simulink model "pd_to_wheel_main"  (R2026a)
settings: Solver=ode45  StopTime=200  MaxStep=0.1
settings Model: Creator=user  LastModifiedBy=user

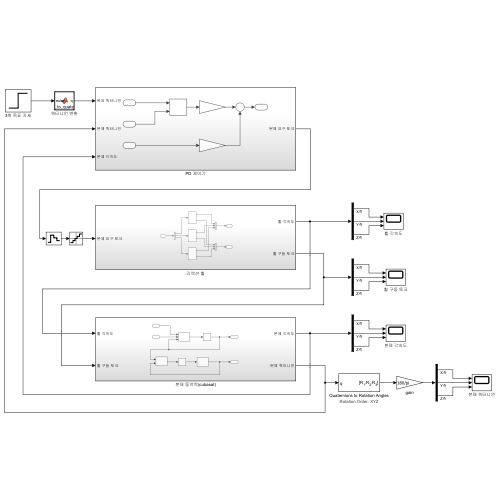
[thumbnail: Simulink's stored preview of the top-level diagram]
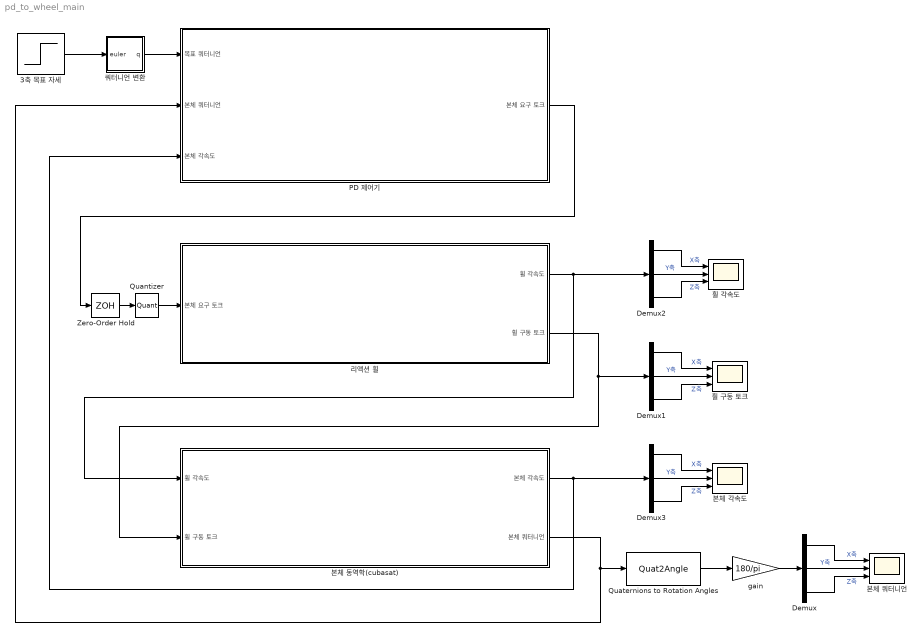
== system pd_to_wheel_main ==
  3축 목표 자세 : Step  InitialValue=[0 0 0]  FinalValue=[5 7 10]*pi/180  SampleTime=0
  Demux{,1..3} (4 alike) : Demux  Outputs=3
  PD 제어기 : Subsystem
  Quantizer : Quantizer  QuantizationInterval=1e-6
  Quaternions to Rotation Angles : Quat2Angle  rotationOrder=XYZ
      settings: AttributesFormatString=Rotation Order: %<rotationOrder>
  Zero-Order Hold : ZeroOrderHold  SampleTime=0.2
  gain : Gain  Gain=180/pi
  리액션 휠 : Subsystem
  본체 각속도 : Scope  NumInputPorts=3
      settings: Title=본체 각속도  ActiveDisplayYMinimum=-0.0017526510151267547  ActiveDisplayYMaximum=0.013773859136141228  DataLoggingVariableName=ScopeData2
  본체 동역학(cubasat) : Subsystem
  본체 쿼터니언 : Scope  NumInputPorts=3
      settings: Title=본체 쿼터니언  ActiveDisplayYMinimum=-1.2703380889069451  ActiveDisplayYMaximum=11.433042800162507
  쿼터니언 변환 : MATLAB Function  TreatAsAtomicUnit=on
  휠 각속도 : Scope  NumInputPorts=3
      settings: Title=휠 가속도  ActiveDisplayYMinimum=-126.21690123764748  ActiveDisplayYMaximum=16.06955468297053
  휠 구동 토크 : Scope  NumInputPorts=3
      settings: Title=휠 구동 토크  ActiveDisplayYMinimum=-0.000403851479395905  ActiveDisplayYMaximum=0.000120427912021545  DataLoggingVariableName=ScopeData3
  wires:
  Zero-Order Hold/1 -> Quantizer/1
  PD 제어기/1(본체 요구 토크) -> Zero-Order Hold/1
  리액션 휠/2(휠 구동 토크) -> Demux1/1, 본체 동역학(cubasat)/2(휠 구동 토크)
  본체 동역학(cubasat)/1(본체 각속도) -> Demux3/1, PD 제어기/3(본체 각속도)
  본체 동역학(cubasat)/2(본체 쿼터니언) -> Quaternions to Rotation Angles/1, PD 제어기/2(본체 쿼터니언)
  Quantizer/1 -> 리액션 휠/1(본체 요구 토크)
  3축 목표 자세/1 -> 쿼터니언 변환/1(euler)
  쿼터니언 변환/1(q) -> PD 제어기/1(목표 쿼터니언)
  리액션 휠/1(휠 각속도) -> Demux2/1, 본체 동역학(cubasat)/1(휠 각속도)
  Quaternions to Rotation Angles/1 -> gain/1
  gain/1 -> Demux/1
  Demux/1 -> 본체 쿼터니언/1  "X축"
  Demux/2 -> 본체 쿼터니언/2  "Y축"
  Demux/3 -> 본체 쿼터니언/3  "Z축"
  Demux1/3 -> 휠 구동 토크/3  "Z축"
  Demux1/2 -> 휠 구동 토크/2  "Y축"
  Demux1/1 -> 휠 구동 토크/1  "X축"
  Demux2/1 -> 휠 각속도/1  "X축"
  Demux2/2 -> 휠 각속도/2  "Y축"
  Demux2/3 -> 휠 각속도/3  "Z축"
  Demux3/3 -> 본체 각속도/3  "Z축"
  Demux3/2 -> 본체 각속도/2  "Y축"
  Demux3/1 -> 본체 각속도/1  "X축"

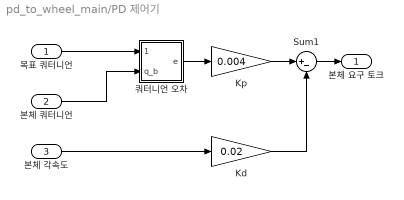
== system pd_to_wheel_main/PD 제어기 ==
  목표 쿼터니언 : Inport  PortDimensions=4
  본체 쿼터니언 : Inport  Port=2  PortDimensions=4
  본체 각속도 : Inport  Port=3  PortDimensions=3
  Kd : Gain  Gain=0.02
  Kp : Gain  Gain=0.004
  Sum1 : Sum  Inputs=|+-
  쿼터니언 오차 : MATLAB Function  TreatAsAtomicUnit=on
  본체 요구 토크 : Outport  PortDimensions=3
  wires:
  Kd/1 -> Sum1/2
  Kp/1 -> Sum1/1
  본체 각속도/1 -> Kd/1
  Sum1/1 -> 본체 요구 토크/1
  쿼터니언 오차/1(e) -> Kp/1
  목표 쿼터니언/1 -> 쿼터니언 오차/1(q_ref)
  본체 쿼터니언/1 -> 쿼터니언 오차/2(q_b)

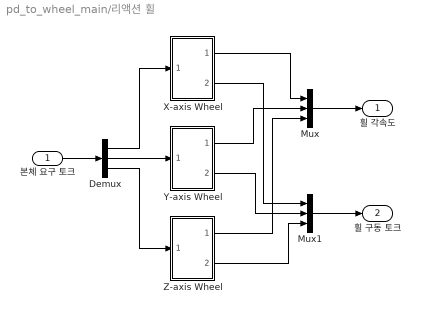
== system pd_to_wheel_main/리액션 휠 ==
  본체 요구 토크 : Inport
  Demux : Demux  Outputs=3
  Mux : Mux  Inputs=3
  Mux1 : Mux  Inputs=3
  X-axis Wheel : Subsystem
  Y-axis Wheel : Subsystem
  Z-axis Wheel : Subsystem
  휠 각속도 : Outport
  휠 구동 토크 : Outport  Port=2
  wires:
  본체 요구 토크/1 -> Demux/1
  Demux/1 -> X-axis Wheel/1(In1)
  Demux/2 -> Y-axis Wheel/1(In1)
  Demux/3 -> Z-axis Wheel/1(In1)
  X-axis Wheel/1(휠 각속도) -> Mux/1
  Y-axis Wheel/1(휠 각속도) -> Mux/2
  Z-axis Wheel/1(휠 각속도) -> Mux/3
  X-axis Wheel/2(휠 구동 토크) -> Mux1/1
  Y-axis Wheel/2(휠 구동 토크) -> Mux1/2
  Z-axis Wheel/2(휠 구동 토크) -> Mux1/3
  Mux/1 -> 휠 각속도/1
  Mux1/1 -> 휠 구동 토크/1

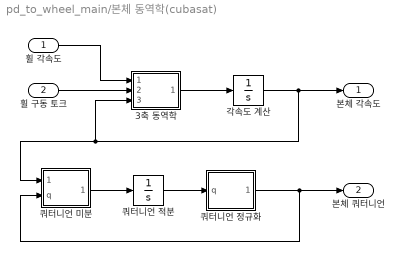
== system pd_to_wheel_main/본체 동역학(cubasat) ==
  휠 각속도 : Inport  PortDimensions=3
  휠 구동 토크 : Inport  Port=2  PortDimensions=3
  3축 동역학 : MATLAB Function  TreatAsAtomicUnit=on
  각속도 계산 : Integrator  InitialCondition=[0;0;0]
  쿼터니언 미분 : MATLAB Function  TreatAsAtomicUnit=on
  쿼터니언 적분 : Integrator  InitialCondition=[1;0;0;0]
  쿼터니언 정규화 : MATLAB Function  TreatAsAtomicUnit=on
  본체 각속도 : Outport  PortDimensions=3
  본체 쿼터니언 : Outport  Port=2  PortDimensions=4
  wires:
  각속도 계산/1 -> 본체 각속도/1, 3축 동역학/3(omega_b), 쿼터니언 미분/1(omega_b)
  휠 각속도/1 -> 3축 동역학/1(omega_w)
  휠 구동 토크/1 -> 3축 동역학/2(tau_w)
  3축 동역학/1(omega_dot) -> 각속도 계산/1
  쿼터니언 미분/1(q_dot) -> 쿼터니언 적분/1
  쿼터니언 적분/1 -> 쿼터니언 정규화/1(q)
  쿼터니언 정규화/1(q_out) -> 쿼터니언 미분/2(q), 본체 쿼터니언/1

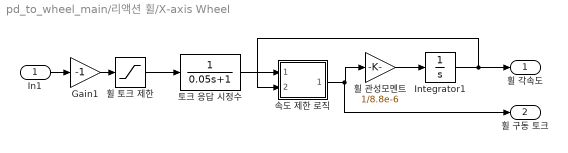
== system pd_to_wheel_main/리액션 휠/X-axis Wheel ==
  In1 : Inport
  Gain1 : Gain  Gain=-1
  Integrator1 : Integrator  LimitOutput=on  UpperSaturationLimit=6000*2*pi/60  LowerSaturationLimit=-6000*2*pi/60
  속도 제한 로직 : MATLAB Function  TreatAsAtomicUnit=on
  토크 응답 시정수 : TransferFcn  Denominator=[0.05 1]
  휠 관성모멘트 : Gain  Gain=1/8.8e-6
  휠 토크 제한 : Saturate  UpperLimit=0.001  LowerLimit=-0.001
  휠 각속도 : Outport
  휠 구동 토크 : Outport  Port=2
  wires:
  Integrator1/1 -> 휠 각속도/1, 속도 제한 로직/2(omega_w)
  Gain1/1 -> 휠 토크 제한/1
  휠 토크 제한/1 -> 토크 응답 시정수/1
  토크 응답 시정수/1 -> 속도 제한 로직/1(tau_in)
  휠 관성모멘트/1 -> Integrator1/1
  속도 제한 로직/1(tau_out) -> 휠 구동 토크/1, 휠 관성모멘트/1
  In1/1 -> Gain1/1

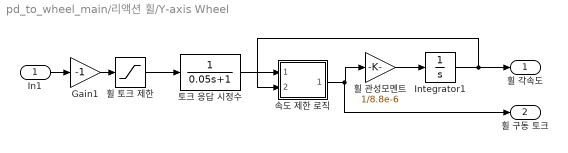
== system pd_to_wheel_main/리액션 휠/Y-axis Wheel ==
  In1 : Inport
  Gain1 : Gain  Gain=-1
  Integrator1 : Integrator  LimitOutput=on  UpperSaturationLimit=6000*2*pi/60  LowerSaturationLimit=-6000*2*pi/60
  속도 제한 로직 : MATLAB Function  TreatAsAtomicUnit=on
  토크 응답 시정수 : TransferFcn  Denominator=[0.05 1]
  휠 관성모멘트 : Gain  Gain=1/8.8e-6
  휠 토크 제한 : Saturate  UpperLimit=0.001  LowerLimit=-0.001
  휠 각속도 : Outport
  휠 구동 토크 : Outport  Port=2
  wires:
  Integrator1/1 -> 휠 각속도/1, 속도 제한 로직/2(omega_w)
  Gain1/1 -> 휠 토크 제한/1
  휠 토크 제한/1 -> 토크 응답 시정수/1
  토크 응답 시정수/1 -> 속도 제한 로직/1(tau_in)
  휠 관성모멘트/1 -> Integrator1/1
  속도 제한 로직/1(tau_out) -> 휠 구동 토크/1, 휠 관성모멘트/1
  In1/1 -> Gain1/1

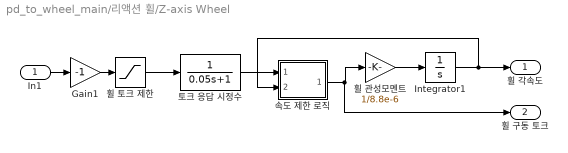
== system pd_to_wheel_main/리액션 휠/Z-axis Wheel ==
  In1 : Inport
  Gain1 : Gain  Gain=-1
  Integrator1 : Integrator  LimitOutput=on  UpperSaturationLimit=6000*2*pi/60  LowerSaturationLimit=-6000*2*pi/60
  속도 제한 로직 : MATLAB Function  TreatAsAtomicUnit=on
  토크 응답 시정수 : TransferFcn  Denominator=[0.05 1]
  휠 관성모멘트 : Gain  Gain=1/8.8e-6
  휠 토크 제한 : Saturate  UpperLimit=0.001  LowerLimit=-0.001
  휠 각속도 : Outport
  휠 구동 토크 : Outport  Port=2
  wires:
  Integrator1/1 -> 휠 각속도/1, 속도 제한 로직/2(omega_w)
  Gain1/1 -> 휠 토크 제한/1
  휠 토크 제한/1 -> 토크 응답 시정수/1
  토크 응답 시정수/1 -> 속도 제한 로직/1(tau_in)
  휠 관성모멘트/1 -> Integrator1/1
  속도 제한 로직/1(tau_out) -> 휠 구동 토크/1, 휠 관성모멘트/1
  In1/1 -> Gain1/1

== matlab function pd_to_wheel_main/리액션 휠/Y-axis Wheel/속도 제한 로직 ==
  data: tau_in input; tau_out output; omega_w input
function tau_out = wheel_speed_limit(tau_in, omega_w)
% Wheel speed saturation test
% tau_in  : Wheel torque [Nm]
% omega_w : Wheel angular velocity [rad/s]

omega_max = 6000 * 2*pi / 60;

tau_out = tau_in;

if omega_w >= omega_max && tau_in > 0
    tau_out = 0;
elseif omega_w <= -omega_max && tau_in < 0
    tau_out = 0;
end
end

== matlab function pd_to_wheel_main/PD 제어기/쿼터니언 오차 ==
  data: q_ref input; e output; q_b input
function e = quaternion_error(q_ref, q_b)
% Scalar-first quaternion: [qw; qx; qy; qz]
% Body-frame attitude error

qr = q_ref(:) / norm(q_ref);
qb = q_b(:) / norm(q_b);

% q_error = conjugate(q_b) * q_ref
a = qb(1);
u = -qb(2:4);

b = qr(1);
v = qr(2:4);

e_scalar = a*b - dot(u,v);
e_vector = a*v + b*u + cross(u,v);

% Shortest rotation
if e_scalar < 0
    e_vector = -e_vector;
end

e = e_vector;
end

== matlab function pd_to_wheel_main/리액션 휠/X-axis Wheel/속도 제한 로직 ==
  data: tau_in input; tau_out output; omega_w input
function tau_out = wheel_speed_limit(tau_in, omega_w)
% Wheel speed saturation test
% tau_in  : Wheel torque [Nm]
% omega_w : Wheel angular velocity [rad/s]

omega_max = 6000 * 2*pi / 60;

tau_out = tau_in;

if omega_w >= omega_max && tau_in > 0
    tau_out = 0;
elseif omega_w <= -omega_max && tau_in < 0
    tau_out = 0;
end
end

== matlab function pd_to_wheel_main/리액션 휠/Z-axis Wheel/속도 제한 로직 ==
  data: tau_in input; tau_out output; omega_w input
function tau_out = wheel_speed_limit(tau_in, omega_w)
% Wheel speed saturation test
% tau_in  : Wheel torque [Nm]
% omega_w : Wheel angular velocity [rad/s]

omega_max = 6000 * 2*pi / 60;

tau_out = tau_in;

if omega_w >= omega_max && tau_in > 0
    tau_out = 0;
elseif omega_w <= -omega_max && tau_in < 0
    tau_out = 0;
end
end

== matlab function pd_to_wheel_main/본체 동역학(cubasat)/3축 동역학 ==
  data: omega_w input; omega_dot output; tau_w input; omega_b input
function omega_dot = body_dynamics(omega_w, tau_w, omega_b)
% omega_w : 휠 각속도 [3x1, rad/s]
% tau_w   : 휠 구동 토크 [3x1, Nm]
% omega_b : 본체 각속도 [3x1, rad/s]

J = diag([0.08 0.08 0.08]);  % 임시 관성행렬
Jw = 8.8e-6;

% 휠 각운동량
h_w = Jw * omega_w;

% 본체 반작용 토크
tau_b = -tau_w;

% 3축 회전 동역학
omega_dot = J \ (tau_b - cross(omega_b, J*omega_b + h_w));
end

== matlab function pd_to_wheel_main/본체 동역학(cubasat)/쿼터니언 미분 ==
  data: omega_b input; q input; q_dot output
function q_dot = quaternion_derivative(omega_b, q)
% q = [qw; qx; qy; qz]
% omega_b = [wx; wy; wz]
% Scalar-first, body-to-inertial quaternion

w = q(1);
v = q(2:4);

q_dot = 0.5 * [-dot(v, omega_b);
                w*omega_b + cross(v, omega_b)];
end

== matlab function pd_to_wheel_main/본체 동역학(cubasat)/쿼터니언 정규화 ==
  data: q input; q_out output
function q_out = normalize_quaternion(q)
q_out = q / norm(q);
end

== matlab function pd_to_wheel_main/쿼터니언 변환 ==
  data: euler input; q output
function q = euler_to_quaternion(euler)
% Rotation order: XYZ
% Input: [Roll; Pitch; Yaw] in radians
% Output: [qw; qx; qy; qz]

roll  = euler(1);
pitch = euler(2);
yaw   = euler(3);

cr = cos(roll/2);
sr = sin(roll/2);
cp = cos(pitch/2);
sp = sin(pitch/2);
cy = cos(yaw/2);
sy = sin(yaw/2);

qw = cr*cp*cy - sr*sp*sy;
qx = sr*cp*cy + cr*sp*sy;
qy = cr*sp*cy - sr*cp*sy;
qz = cr*cp*sy + sr*sp*cy;

q = [qw; qx; qy; qz];
end
